simulink model "simulation"  (R2026b)
settings: Solver=ode23s  StopTime=T_sim  MaxStep=1e-3  MinStep=1e-7  RelTol=1e-5
InitFcn:
  | run param_file.m
values from neighbouring files (symbols this model uses):
  param = struct()    [param_file.m]    (also in param_file_2.m)
settings Model: Creator=user  LastModifiedBy=mahmu
settings SolverCC: ZeroCrossAlgorithm=Adaptive
settings DebuggingCC: IgnoredZcDiagnostic=none
settings SimscapeCC: SimscapeUseEnergyAccounting=off

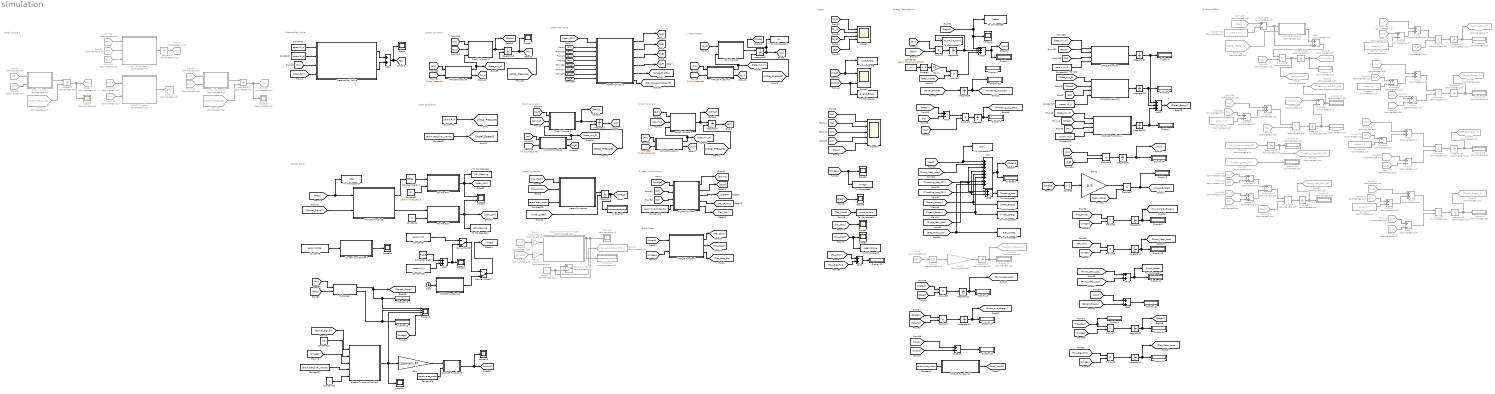
== system simulation ==
  note: Hydraulic Effort
  note: Small Volume A
  note: Control Policy
  note: BLDC Motor
  note: Energy Calculations
  note: Pressure Rail Valve
  note: Scope
  note: Initial Conditions
  note: Hydraulic Motor/Pump
  note: Inertia Dynamics
  note: Small Volume T
  note: Small Volume P
  note: Soft-Switch Valve
  note: Linear Actuator
  note: Small Voume A
  Add : Sum  Inputs=++++++++
  Add1 : Sum  Inputs=+-
  Add{10,12..13,15,17..18} (6 alike) : Sum  Commented=on
  Add11 : Sum  Commented=on  Inputs=+-
  Add14 : Sum  Commented=on  Inputs=+-
  Add16 : Sum  Commented=on  Inputs=+-
  Add2 : Sum  Inputs=+++
  Add{3..7,9} (6 alike) : Sum
  Add8 : Sum  Inputs=+++
  Clock : Clock
  Constant{,12,14..17} (6 alike) : Constant  Commented=on  Value=param.P_T
  Constant1 : Constant  Value=param.P_M
  Constant10 : Constant
  Constant11 : Constant  Value=15
  Constant13 : Constant  Value=param.P_M
  Constant18 : Constant  Value=param.VA_0
  Constant19 : Constant  Value=param.VP_0
  Constant2 : Constant  Value=param.P_H
  Constant20 : Constant  Value=param.VT_0
  Constant21 : Constant  Value=param.start_final_velocity
  Constant22 : Constant  Value=param.start_final_velocity
  Constant23 : Constant  Value=param.hyd_motor_fric
  Constant24 : Constant  Commented=on  Value=0
  Constant25 : Constant  Value=param.elec_motor
  Constant26 : Constant  Value=param.elec_motor
  Constant3 : Constant  Value=param.start_final_velocity
  Constant4 : Constant  Value=param.elec_motor
  Constant5 : Constant  Value=param.initial_stroke
  Constant6 : Constant  Value=0
  Constant7 : Constant  Value=param.P_M
  Constant8 : Constant  Value=param.stroke
  Constant9 : Constant  Value=param.P_H
  Display{,1..20,32,35..36} (24 alike) : Display
  Display{21..31,34} (12 alike) : Display  Commented=on
  Dynamics of Orifice 3 : Subsystem
  Electric Torque Controller1 : MATLAB Function  TreatAsAtomicUnit=on
  Experimental Friction Model : MATLAB Function  Commented=on  TreatAsAtomicUnit=on
  For the PRV : Subsystem
  For the SSV : Subsystem
  From : From  Commented=on  GotoTag=Initial_Pressure
  From100 : From  Commented=on  GotoTag=Q_A
  From{6,97,99,104} (4 alike) : From  Commented=on  GotoTag=Qh1
  From105 : From  Commented=on  GotoTag=Ph1
  From{98,106,113,133} (4 alike) : From  Commented=on  GotoTag=PA
  From112 : From  Commented=on  GotoTag=W_A
  From{21,114,134,168} (4 alike) : From  Commented=on  GotoTag=Q1
  From115 : From  Commented=on  GotoTag=Q_A
  From116 : From  Commented=on  GotoTag=Q_B
  From117 : From  Commented=on  GotoTag=PX
  From118 : From  Commented=on  GotoTag=W_X
  From119 : From  Commented=on  GotoTag=W_P
  From120 : From  Commented=on  GotoTag=PP
  From121 : From  Commented=on  GotoTag=Q_P
  From122 : From  Commented=on  GotoTag=Qpump
  From123 : From  Commented=on  GotoTag=PT
  From124 : From  Commented=on  GotoTag=W_T
  From125 : From  Commented=on  GotoTag=Pdes
  From126 : From  Commented=on  GotoTag=Qpump
  From127 : From  Commented=on  GotoTag=Q_T
  From128 : From  Commented=on  GotoTag=Input_HE
  From130 : From  Commented=on  GotoTag=W_A
  From131 : From  Commented=on  GotoTag=Initial_Pressure
  From135 : From  Commented=on  GotoTag=Throttling_Loss_SSV
  From140 : From  Commented=on  GotoTag=SSV_Power_throttle_HE
  From15 : From  Commented=on  GotoTag=PX
  From150 : From  Commented=on  GotoTag=Qleak
  From151 : From  Commented=on  GotoTag=PT
  From152 : From  Commented=on  GotoTag=PP
  From153 : From  Commented=on  GotoTag=W_P
  From154 : From  Commented=on  GotoTag=W_T
  From16 : From  Commented=on  GotoTag=omega
  From19 : From  Commented=on  GotoTag=Initial_Pressure
  From96 : From  Commented=on  GotoTag=Ph1
  Gain : Gain  Gain=1/param.Kt
  Gain1 : Gain  Gain=0.5
  Gain2 : Gain  Commented=on  Gain=0.000145038
  Gain3 : Gain  Commented=on  Gain=(60/(2*pi))
  Gain5 : Gain  Gain=0.5
  Gain6 : Gain  Commented=on  Gain=param.ResistHose
  Goto2 : Goto  Commented=on  GotoTag=Ph1
  Goto22 : Goto  Commented=on  GotoTag=experimental_friction
  Goto39 : Goto  Commented=on  GotoTag=PA
  Goto40 : Goto  Commented=on  GotoTag=Hose_Throttle_Loss
  Goto41 : Goto  Commented=on  GotoTag=Qh1
  Goto42 : Goto  Commented=on  GotoTag=Qh1
  Goto48 : Goto  Commented=on  GotoTag=Input_HE
  Goto49 : Goto  Commented=on  GotoTag=Stored_Energy_A
  Goto51 : Goto  Commented=on  GotoTag=Throttling_Loss_PRV_HE
  Goto52 : Goto  Commented=on  GotoTag=Throttling_Loss_SSV_HE
  Goto53 : Goto  Commented=on  GotoTag=Output_Energy
  Goto54 : Goto  Commented=on  GotoTag=Stored_Energy_P
  Goto55 : Goto  Commented=on  GotoTag=Stored_Energy_T
  Goto56 : Goto  Commented=on  GotoTag=Pump_Leak_Loss_HE
  Goto57 : Goto  Commented=on  GotoTag=Input_Power
  Hydraulic Motor : MATLAB Function  TreatAsAtomicUnit=on
  Inertia Dynamics : MATLAB Function  TreatAsAtomicUnit=on
  Integrator : Integrator  Commented=on  InitialConditionSource=external
  Integrator{1..4,18} (5 alike) : Integrator  InitialConditionSource=external
  Integrator{5,7..14,27..29,31} (13 alike) : Integrator
  Integrator{15,17,19..26} (10 alike) : Integrator  Commented=on
  Integrator16 : Integrator  Commented=on  InitialConditionSource=external
  MATLAB Function : MATLAB Function  TreatAsAtomicUnit=on
  MATLAB Function1 : MATLAB Function  TreatAsAtomicUnit=on
  MATLAB Function10 : MATLAB Function  TreatAsAtomicUnit=on
  MATLAB Function11 : MATLAB Function  TreatAsAtomicUnit=on
  MATLAB Function12 : MATLAB Function  TreatAsAtomicUnit=on
  MATLAB Function13 : MATLAB Function  TreatAsAtomicUnit=on
  MATLAB Function14 : MATLAB Function  TreatAsAtomicUnit=on
  MATLAB Function2 : MATLAB Function  Commented=on  TreatAsAtomicUnit=on
  MATLAB Function3 : MATLAB Function  TreatAsAtomicUnit=on
  MATLAB Function4 : MATLAB Function  Commented=on  TreatAsAtomicUnit=on
  MATLAB Function5 : MATLAB Function  TreatAsAtomicUnit=on
  MATLAB Function6 : MATLAB Function  TreatAsAtomicUnit=on
  MATLAB Function7 : MATLAB Function  TreatAsAtomicUnit=on
  MATLAB Function8 : MATLAB Function  TreatAsAtomicUnit=on
  MATLAB Function9 : MATLAB Function  Commented=on  TreatAsAtomicUnit=on
  Main Chamber : MATLAB Function  TreatAsAtomicUnit=on
  Manual Switch : ManualSwitch  CurrentSetting=0
  Manual Switch2 : ManualSwitch  CurrentSetting=0
  Manual Switch3 : ManualSwitch  Commented=on  CurrentSetting=0
  Pressure Rail Valve : MATLAB Function  TreatAsAtomicUnit=on
  Product{,1..8,16..17} (11 alike) : Product
  Product{9..15} (7 alike) : Product  Commented=on
  Pulse Generator : DiscretePulseGenerator  PulseType=Time based  Amplitude=param.P_H-param.P_M  Period=param.T_period  PulseWidth=50  PhaseDelay=param.delay
  Scope{,5..8,10..12,14..15,17} (11 alike) : Scope
      Scope settings: ActiveDisplayYMinimum=-7.8990948168927051E-6  ActiveDisplayYMaximum=6.46174239346027E-5  DataLoggingVariableName=ScopeData14
      Scope10 settings: ActiveDisplayYMinimum=-1  ActiveDisplayYMaximum=1  DataLoggingVariableName=ScopeData9
      Scope11 settings: ActiveDisplayYMinimum=-0.9375  ActiveDisplayYMaximum=0.9375  DataLoggingVariableName=ScopeData10
      Scope12 settings: ActiveDisplayYMinimum=-1  ActiveDisplayYMaximum=1  DataLoggingVariableName=ScopeData11
      Scope14 settings: ActiveDisplayYMinimum=-2.6515706692780068  ActiveDisplayYMaximum=0.29461896325311182  DataLoggingVariableName=ScopeData13
      Scope15 settings: ActiveDisplayYMinimum=-1  ActiveDisplayYMaximum=1  DataLoggingVariableName=ScopeData15
      Scope17 settings: ActiveDisplayYMinimum=2.5851457116932129E+6  ActiveDisplayYMaximum=1.1203688594761087E+7  DataLoggingVariableName=ScopeData17
      Scope5 settings: ActiveDisplayYMinimum=-714867.26768483547  ActiveDisplayYMaximum=268797.57913288096  DataLoggingVariableName=ScopeData3
      Scope6 settings: ActiveDisplayYMinimum=-2.1163885820684094E-7  ActiveDisplayYMaximum=1.4152197079471591E-6  DataLoggingVariableName=ScopeData5
      Scope7 settings: ActiveDisplayYMinimum=-1.2648949471331186  ActiveDisplayYMaximum=0.69609943857034651  DataLoggingVariableName=ScopeData6
      Scope8 settings: ActiveDisplayYMinimum=-1  ActiveDisplayYMaximum=1  DataLoggingVariableName=ScopeData7
  Scope1 : Scope  NumInputPorts=4
      settings: ActiveDisplayYMinimum=-0.00094060960760663083  ActiveDisplayYMaximum=0.00094060960760663083
  Scope13 : Scope  NumInputPorts=4
      settings: ActiveDisplayYMinimum=-0.12499999999999997  ActiveDisplayYMaximum=1.125  DataLoggingVariableName=ScopeData12
  Scope16 : Scope  Commented=on
      settings: ActiveDisplayYMinimum=2.3595705734494529E+6  ActiveDisplayYMaximum=1.140070781407249E+7  DataLoggingVariableName=ScopeData16
  Scope18 : Scope  Commented=on
      settings: ActiveDisplayYMinimum=2.6611575254358238E+8  ActiveDisplayYMaximum=4.6611575254358238E+8  DataLoggingVariableName=ScopeData18
  Scope2 : Scope  NumInputPorts=2
      settings: ActiveDisplayYMinimum=0.33341582524675561  ActiveDisplayYMaximum=8.9612181068995049
  Scope3 : Scope  NumInputPorts=5
      settings: ActiveDisplayYMinimum=1.6778033246308342E+6  ActiveDisplayYMaximum=1.9369768489858452E+7  DataLoggingVariableName=ScopeData2
  Scope4 : Scope  Commented=on
      settings: ActiveDisplayYMinimum=2.181490968537122E+6  ActiveDisplayYMaximum=1.1231186415855616E+7  DataLoggingVariableName=ScopeData4
  Scope9 : Scope  NumInputPorts=2
      settings: ActiveDisplayYMinimum=-2.9871968388761352  ActiveDisplayYMaximum=1.7269260169317651  DataLoggingVariableName=ScopeData8
  Small Volume A : MATLAB Function  Commented=on  TreatAsAtomicUnit=on
  Small Volume A1 : MATLAB Function  Commented=on  TreatAsAtomicUnit=on
  Small Volume A2 : MATLAB Function  TreatAsAtomicUnit=on
  Small Volume P : MATLAB Function  TreatAsAtomicUnit=on
  Small Volume T : MATLAB Function  TreatAsAtomicUnit=on
  Soft-switch Valve : MATLAB Function  TreatAsAtomicUnit=on
  Square : Math  Commented=on  Operator=square
  Square1 : Math  Operator=square
  Square5 : Math  Operator=square
  Subsystem : Subsystem
  Subtract : Sum  Inputs=+-
  Subtract{3,6..11,14} (8 alike) : Sum  Commented=on  Inputs=+-
  Subtract12 : Sum  Commented=on
  Subtract13 : Sum  Commented=on
  To Workspace : ToWorkspace  VariableName=Input_Energy  SaveFormat=Timeseries  SampleTime=-1
  To Workspace1 : ToWorkspace  VariableName=Output_Energy  SaveFormat=Timeseries  SampleTime=-1
  To Workspace10 : ToWorkspace  VariableName=PRV_Opening  SaveFormat=Timeseries  SampleTime=-1
  To Workspace11 : ToWorkspace  VariableName=SSV_Opening  SaveFormat=Timeseries  SampleTime=-1
  To Workspace12 : ToWorkspace  VariableName=Hydraulic_Input  SaveFormat=Timeseries  SampleTime=-1
  To Workspace13 : ToWorkspace  VariableName=Px  SaveFormat=Timeseries  SampleTime=-1
  To Workspace14 : ToWorkspace  VariableName=Pdes  SaveFormat=Timeseries  SampleTime=-1
  To Workspace15 : ToWorkspace  VariableName=regen_torque  SaveFormat=Timeseries  SampleTime=-1
  To Workspace16 : ToWorkspace  VariableName=pump_torque  SaveFormat=Timeseries  SampleTime=-1
  To Workspace2 : ToWorkspace  VariableName=Work  SaveFormat=Timeseries  SampleTime=-1
  To Workspace3 : ToWorkspace  VariableName=Throttling_Loss  SaveFormat=Timeseries  SampleTime=-1
  To Workspace4 : ToWorkspace  VariableName=Stored_Energy  SaveFormat=Timeseries  SampleTime=-1
  To Workspace5 : ToWorkspace  VariableName=Kinetic_Energy  SaveFormat=Timeseries  SampleTime=-1
  To Workspace6 : ToWorkspace  VariableName=omega  SaveFormat=Timeseries  SampleTime=-1
  To Workspace7 : ToWorkspace  VariableName=Pump_Losses  SaveFormat=Timeseries  SampleTime=-1
  To Workspace8 : ToWorkspace  VariableName=Elec_Losses  SaveFormat=Timeseries  SampleTime=-1
  To Workspace9 : ToWorkspace  VariableName=Regen  SaveFormat=Timeseries  SampleTime=-1
  Transport Delay2 : TransportDelay  DelayTime=param.delay_switch  InitialOutput=param.initial_stroke  BufferSize=1024*105
  wires:
  Constant2/1 -> Pressure Rail Valve/1(P)
  Small Volume A/1(Ph1dot) -> Integrator/1
  Constant1/1 -> [Initial_Pressure]
  From/1 -> Integrator/2
  Integrator/1 -> Goto2/1, Scope4/1  "PA"
  Small Volume P/1(PPdot) -> [PPdot], Integrator1/1
  [Initial_Pressure] -> Integrator1/2
  Small Volume T/1(PTdot) -> [PTdot], Integrator2/1
  [Initial_Pressure] -> Integrator2/2
  Main Chamber/1(PXdot) -> Integrator3/1
  [Initial_Pressure] -> Integrator3/2
  Integrator3/1 -> [PX], [PXdot], To Workspace13/1  "PX"
  [PA] -> Soft-switch Valve/3(PA)
  [omega] -> Hydraulic Motor/1(omega)
  Integrator1/1 -> [PP]  "PP"
  Integrator2/1 -> [PT]  "PT"
  [PP] -> Soft-switch Valve/2(PP)
  [PT] -> Soft-switch Valve/5(PT)
  [PX] -> Soft-switch Valve/4(PB)
  Soft-switch Valve/4(Q_T) -> [Q_T]  "Q_T"
  Soft-switch Valve/3(Q_B) -> [Q_B]  "Q_B"
  Soft-switch Valve/2(Q_A) -> [Q_A]  "Q_A"
  [Q_T] -> Small Volume T/1(QT)
  Hydraulic Motor/1(Qpump) -> [Qpump]
  [Qpump] -> Small Volume T/2(Qpump)
  [Qpump] -> Small Volume P/2(Qpump)
  [Q_P] -> Small Volume P/1(QP)
  [Q_B] -> Main Chamber/1(QB)
  From99/1 -> Small Volume A/2(Qh1)
  Constant22/1 -> [Initial_Speed]
  From21/1 -> Small Volume A/1(Q1)
  [Q_P] -> Scope1/1
  [Q_A] -> Scope1/2
  [Q_B] -> Scope1/3
  [Q_T] -> Scope1/4
  [Q1] -> Product/1
  [Pdes] -> Product/2
  Product/1 -> Integrator5/1
  [Work] -> To Workspace2/1, Add/1
  [Kinetic_Energy] -> To Workspace5/1, Add/6
  Add/1 -> Display3/1, [Output]
  [PA] -> Add1/2
  Add1/1 -> Product2/1
  [Q1] -> Product2/2
  Product2/1 -> Integrator7/1
  Integrator7/1 -> [Throttling_Loss_PRV], Display4/1
  [Throttling_Loss_PRV] -> Add3/1, Add/3
  Soft-switch Valve/1(Q_P) -> [Q_P]  "Q_P"
  Soft-switch Valve/5(Power_throttle) -> [Power_throttle]
  Integrator27/1 -> Display6/1, Add2/1
  Integrator28/1 -> Add2/2, Display2/1
  Square5/1 -> Gain5/1
  [omega] -> Square5/1
  [Stored_Energy] -> To Workspace4/1, Add/5
  Add2/1 -> [Stored_Energy]
  [Input] -> Scope2/1, To Workspace/1  "Input"
  [Output] -> To Workspace1/1, Scope2/2  "Output"
  Integrator8/1 -> Display35/1, [Throttling_Loss_SSV]
  [Throttling_Loss_SSV] -> Add3/2, Add/4
  Add3/1 -> To Workspace3/1
  [PX] -> Scope3/4
  [omega] -> Product3/2
  [Tau_Pump] -> Product3/1
  Integrator9/1 -> [Pump_Mech_Energy], Display9/1
  Product3/1 -> Integrator9/1
  Hydraulic Motor/3(DeltaP) -> [DeltaP]
  [DeltaP] -> Product4/1
  [Qpump] -> Product4/2
  Product4/1 -> Integrator10/1
  Integrator10/1 -> [Pump_Hyd_Energy], Display10/1
  [omega] -> To Workspace6/1, Scope5/1
  Hydraulic Motor/2(Qleak) -> [Qleak]
  [Qleak] -> Scope6/1
  [PT] -> Hydraulic Motor/2(PT)
  [PP] -> Hydraulic Motor/3(PP)
  [DeltaP] -> Product5/1
  [Qleak] -> Product5/2
  Product5/1 -> Integrator11/1
  Integrator11/1 -> [Pump_Leak_Loss], Display11/1
  [Pump_Mech_Loss] -> Add/2
  [Tau_fric] -> Product6/1
  [omega] -> Product6/2
  Product6/1 -> Integrator12/1
  Integrator12/1 -> [Pump_Mech_Loss], Display13/1
  [Pump_Leak_Loss] -> Add/7
  [Pump_Leak_Loss] -> Add5/1
  [Pump_Mech_Loss] -> Add5/2
  Add5/1 -> To Workspace7/1, Display14/1
  [Work] -> Add4/1
  [Stored_Energy] -> Add4/2
  Add4/1 -> Display12/1
  [Pdes] -> Scope3/5
  [PT] -> Scope3/3
  [PP] -> Scope3/2
  [omega] -> MATLAB Function1/2(omega)
  [current] -> MATLAB Function1/1(current)
  MATLAB Function1/1(Tau_Elec) -> [Tau_Elec]
  MATLAB Function1/2(Tau_Mech) -> [Tau_Mech]
  [Tau_Elec] -> Scope7/1
  [Tau_Mech] -> To Workspace15/1, Scope8/1
  For the PRV/1(Spool Opening) -> [open_PRV], To Workspace10/1, Scope9/1
  [Control_Signal] -> MATLAB Function3/2(Control_signal)
  Transport Delay2/1 -> For the PRV/1(Opening)
  MATLAB Function3/1(open_PRV) -> Transport Delay2/1
  MATLAB Function3/2(open_SSV) -> For the SSV/1(Opening)
  Pressure Rail Valve/1(Q_PA) -> Add6/1
  Pressure Rail Valve/2(Q_AT) -> Add6/2
  Add6/1 -> Scope/1, [Q1]
  [PA] -> Pressure Rail Valve/3(PA)
  Constant7/1 -> Pressure Rail Valve/2(T)
  [open_PRV] -> Pressure Rail Valve/4(spool_position)
  [open_SSV] -> Soft-switch Valve/1(spool_position)
  [Pdes] -> Subsystem/2(Pdes)
  [PX] -> Subsystem/1(PX)
  Subsystem/1(Control_Signal) -> [Control_Signal], Scope13/1, Display15/1  "Control Signal"
  Subsystem/2(delP) -> Scope13/2, Display16/1  "delP"
  Manual Switch2/1 -> [Pdes]  "Pdes"
  Constant10/1 -> Electric Torque Controller1/5(T_elec_max)
  Constant9/1 -> Manual Switch/1
  Constant13/1 -> Add7/2
  Pulse Generator/1 -> Add7/1
  Add7/1 -> Manual Switch/2, Scope12/1
  Dynamics of Orifice 3/1(Spool Opening) -> Scope10/1
  Constant8/1 -> Dynamics of Orifice 3/1(Stroke)
  [omega] -> Scope13/4
  [Control_Signal] -> Electric Torque Controller1/1(Control_Signal)
  Electric Torque Controller1/1(T_elec) -> Scope13/3, Gain/1, Scope11/1  "T_elec"
  [Pdes] -> To Workspace14/1, MATLAB Function3/1(Pdes)
  [Tau_Elec] -> Product7/1, Display5/1
  [omega] -> Product7/2
  Product7/1 -> Integrator13/1
  Integrator13/1 -> [Regen], Display17/1
  [Input] -> Subtract/1  "Input"
  [Output] -> Subtract/2  "Output"
  Subtract/1 -> Display18/1
  MATLAB Function1/3(Tau_Elec_Fric) -> [Tau_Elec_Fric]
  [Tau_Elec_Fric] -> Product8/1
  [omega] -> Product8/2
  Product8/1 -> Integrator14/1
  Integrator14/1 -> [Elec_Motor_Loss], Display19/1
  [Power_throttle] -> Integrator8/1
  [Pdes] -> Add1/1
  [Regen] -> To Workspace9/1, Add8/1, Scope14/1
  Integrator5/1 -> To Workspace12/1, Add8/2
  Add8/1 -> Display/1, [Input]
  [Elec_Motor_Loss] -> To Workspace8/1, Add/8
  [Initial_Speed] -> Integrator4/2
  Inertia Dynamics/1(omegadot) -> Integrator4/1
  Integrator4/1 -> Display32/1, [omega]  "omega"
  Gain/1 -> MATLAB Function13/1(current_in)
  MATLAB Function13/1(current) -> Scope15/1, [current]
  [Tau_Elec_Fric] -> Add9/2
  [Tau_fric] -> Add9/1
  Add9/1 -> Display20/1
  Constant5/1 -> For the PRV/2(Initial Stroke)
  Constant6/1 -> For the SSV/2(Initial Stroke)
  From6/1 -> Square/1
  Square/1 -> Gain6/1
  Gain6/1 -> Integrator15/1
  Integrator16/1 -> Scope16/1, Goto39/1  "PA"
  From19/1 -> Integrator16/2
  Small Volume A1/1(PAdot) -> Integrator16/1
  From97/1 -> Small Volume A1/1(Qh1)
  From100/1 -> Small Volume A1/2(QA)
  From96/1 -> MATLAB Function2/1(Ph1)
  From98/1 -> MATLAB Function2/2(PA)
  Integrator15/1 -> Goto40/1, Display22/1
  MATLAB Function2/1(Qh1dot) -> Integrator17/1
  Integrator17/1 -> Goto41/1
  From104/1 -> MATLAB Function2/3(Qh1)
  From105/1 -> MATLAB Function4/1(Ph1)
  From106/1 -> MATLAB Function4/2(PA)
  MATLAB Function4/1(Qh1) -> Goto42/1
  [Q_A] -> Small Volume A2/2(QA)
  Integrator18/1 -> [PA], Scope17/1  "PA"
  [Initial_Pressure] -> Integrator18/2
  Small Volume A2/1(PAdot) -> [PAdot], Integrator18/1
  MATLAB Function5/1(beta_mix_A) -> Small Volume A2/3(beta_mix), [beta_mix_A]
  [PA] -> MATLAB Function5/1(P)
  [PP] -> MATLAB Function6/1(P)
  MATLAB Function6/1(beta_mix) -> [beta_mix_P], Small Volume P/3(beta_mix)
  [PT] -> MATLAB Function7/1(P)
  MATLAB Function8/1(beta_mix) -> [beta_mix_X], Main Chamber/2(beta_mix)
  [PX] -> MATLAB Function8/1(P)
  MATLAB Function5/2(WA) -> [W_A]
  From113/1 -> Subtract3/1
  Constant/1 -> Subtract3/2
  Integrator19/1 -> Goto49/1, Display23/1
  From112/1 -> Add10/1
  Subtract3/1 -> Add10/2
  Add10/1 -> Product9/1
  Product9/1 -> Integrator19/1
  From115/1 -> Add11/2
  Add11/1 -> Product9/2
  MATLAB Function8/2(WX) -> [W_X]
  From117/1 -> Subtract6/1
  Constant12/1 -> Subtract6/2
  From118/1 -> Add12/1
  Subtract6/1 -> Add12/2
  Add12/1 -> Product10/1
  From116/1 -> Product10/2
  Product10/1 -> Integrator20/1
  Integrator20/1 -> Display24/1, Goto53/1
  MATLAB Function6/2(WP) -> [W_P]
  Constant14/1 -> Subtract8/2
  From120/1 -> Subtract8/1
  From119/1 -> Add13/1
  Subtract8/1 -> Add13/2
  From121/1 -> Add14/1
  From122/1 -> Add14/2
  Add13/1 -> Product11/1
  Add14/1 -> Product11/2
  Product11/1 -> Integrator21/1
  Integrator21/1 -> Goto54/1, Display25/1
  MATLAB Function7/2(WT) -> [W_T]
  Constant15/1 -> Subtract7/2
  From123/1 -> Subtract7/1
  Subtract7/1 -> Add15/2
  From124/1 -> Add15/1
  From126/1 -> Add16/1
  From127/1 -> Add16/2
  Add15/1 -> Product12/1
  Add16/1 -> Product12/2
  Product12/1 -> Integrator22/1
  Integrator22/1 -> Goto55/1, Display26/1
  From125/1 -> Subtract9/1
  Constant16/1 -> Subtract9/2
  MATLAB Function9/1(Win) -> Add17/1
  Subtract9/1 -> Add17/2, MATLAB Function9/1(P)
  Add17/1 -> Product13/1
  Product13/1 -> Goto57/1, Integrator23/1
  Integrator23/1 -> Goto48/1, Display28/1
  From131/1 -> MATLAB Function9/2(P_initial)
  [Initial_Pressure] -> MATLAB Function5/2(P_initial)
  Product14/1 -> Integrator24/1
  Add18/1 -> Product14/1
  Subtract10/1 -> Add18/2
  From130/1 -> Add18/1
  Integrator24/1 -> Subtract11/2, Display27/1
  Constant17/1 -> Subtract10/2
  From133/1 -> Subtract10/1
  From128/1 -> Subtract11/1
  Subtract11/1 -> Goto51/1, Display29/1
  [W_A] -> Soft-switch Valve/6(WA)
  [W_P] -> Soft-switch Valve/7(WP)
  [W_T] -> Soft-switch Valve/9(WT)
  [W_X] -> Soft-switch Valve/8(WB)
  Soft-switch Valve/6(SSV_Power_throttle_HE) -> [SSV_Power_throttle_HE]
  From140/1 -> Integrator25/1
  Integrator25/1 -> Goto52/1, Display30/1
  From135/1 -> Display31/1
  From150/1 -> Product15/2
  Product15/1 -> Integrator26/1
  From153/1 -> Subtract12/1
  From152/1 -> Subtract12/2
  From151/1 -> Subtract13/2
  From154/1 -> Subtract13/1
  Subtract12/1 -> Subtract14/1
  Subtract13/1 -> Subtract14/2
  Subtract14/1 -> Product15/1
  Integrator26/1 -> Goto56/1, Display34/1
  [Initial_Pressure] -> MATLAB Function8/2(P_initial)
  [Initial_Pressure] -> MATLAB Function6/2(P_initial)
  [Initial_Pressure] -> MATLAB Function7/2(P_initial)
  From168/1 -> Product13/2
  [Q1] -> Small Volume A2/1(Q1)
  From114/1 -> Add11/1
  From134/1 -> Product14/2
  [beta_mix_A] -> MATLAB Function/1(beta_mix)
  [PAdot] -> MATLAB Function/2(Pdot)
  [PA] -> MATLAB Function/3(P)
  Constant18/1 -> MATLAB Function/4(Volume)
  MATLAB Function/1(Stored_Power) -> Integrator27/1
  MATLAB Function10/1(Stored_Power) -> Integrator28/1
  [beta_mix_P] -> MATLAB Function10/1(beta_mix)
  [PPdot] -> MATLAB Function10/2(Pdot)
  [PP] -> MATLAB Function10/3(P)
  Constant19/1 -> MATLAB Function10/4(Volume)
  Integrator29/1 -> Add2/3, Display7/1
  MATLAB Function11/1(Stored_Power) -> Integrator29/1
  MATLAB Function7/1(beta_mix) -> [beta_mix_T], Small Volume T/3(beta_mix)
  [beta_mix_T] -> MATLAB Function11/1(beta_mix)
  [PTdot] -> MATLAB Function11/2(Pdot)
  [PT] -> MATLAB Function11/3(P)
  Constant20/1 -> MATLAB Function11/4(Volume)
  [Q_B] -> Product16/2
  [PX] -> Product16/1
  Product16/1 -> Integrator31/1
  Integrator31/1 -> Display36/1, [Work]
  [PA] -> Scope3/1
  [omega] -> Electric Torque Controller1/3(omega)
  Constant11/1 -> Electric Torque Controller1/2(Kp)
  Constant21/1 -> Electric Torque Controller1/4(start_final_velocity)
  Square1/1 -> Gain1/1
  Constant3/1 -> Square1/1
  Hydraulic Motor/4(Tau_Pump) -> [Tau_Pump]
  Hydraulic Motor/5(Tau_Fric) -> [Tau_fric]
  [Tau_Pump] -> Inertia Dynamics/2(Tau_Pump)
  Constant23/1 -> Hydraulic Motor/4(fric)
  Clock/1 -> MATLAB Function12/1(clock_time)
  MATLAB Function12/1(Pdes) -> Manual Switch2/2
  Manual Switch/1 -> Manual Switch2/1
  [Tau_Mech] -> Inertia Dynamics/1(Tau_Mech)
  From15/1 -> Gain2/1
  From16/1 -> Gain3/1
  Experimental Friction Model/1(friction) -> Display21/1, Manual Switch3/1, Scope18/1
  Gain2/1 -> Experimental Friction Model/1(pressure)
  Gain3/1 -> Experimental Friction Model/2(speed)
  Constant24/1 -> Goto22/1, Manual Switch3/2
  For the SSV/1(Spool Opening) -> [open_SSV], To Workspace11/1, Scope9/2
  Constant25/1 -> Inertia Dynamics/4(elec_motor)
  [Tau_Pump] -> To Workspace16/1
  Constant26/1 -> MATLAB Function13/2(elec_motor)
  Constant4/1 -> MATLAB Function14/1(elec_motor)
  MATLAB Function14/1(inertia) -> [total_inertia]
  Gain1/1 -> Product1/1
  [total_inertia] -> Product1/2
  Product1/1 -> Add8/3
  Gain5/1 -> Product17/1
  [total_inertia] -> Product17/2
  Product17/1 -> Display8/1, [Kinetic_Energy]

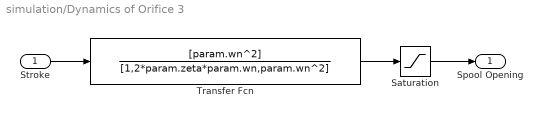
== system simulation/Dynamics of Orifice 3 ==
  Stroke : Inport
  Saturation : Saturate  UpperLimit=param.stroke  LowerLimit=0
  Transfer Fcn : TransferFcn  Numerator=[param.wn^2]  Denominator=[1,2*param.zeta*param.wn,param.wn^2]
  Spool Opening : Outport
  wires:
  Transfer Fcn/1 -> Saturation/1
  Saturation/1 -> Spool Opening/1
  Stroke/1 -> Transfer Fcn/1

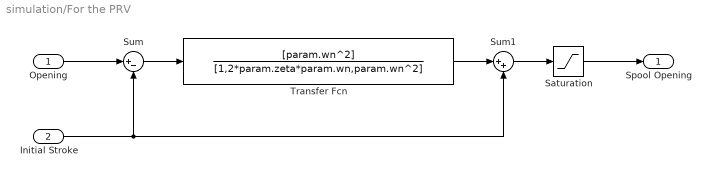
== system simulation/For the PRV ==
  Opening : Inport
  Initial Stroke : Inport  Port=2
  Saturation : Saturate  UpperLimit=1  LowerLimit=-1
  Sum : Sum  Inputs=|+-
  Sum1 : Sum  Inputs=|++
  Transfer Fcn : TransferFcn  Numerator=[param.wn^2]  Denominator=[1,2*param.zeta*param.wn,param.wn^2]
  Spool Opening : Outport
  wires:
  Saturation/1 -> Spool Opening/1
  Sum1/1 -> Saturation/1
  Transfer Fcn/1 -> Sum1/1
  Sum/1 -> Transfer Fcn/1
  Opening/1 -> Sum/1
  Initial Stroke/1 -> Sum1/2, Sum/2

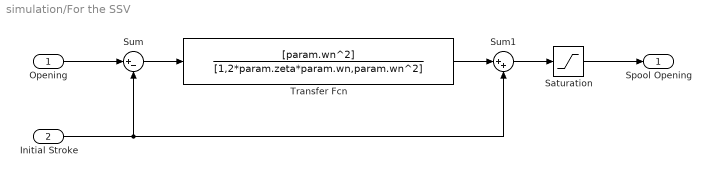
== system simulation/For the SSV ==
  Opening : Inport
  Initial Stroke : Inport  Port=2
  Saturation : Saturate  UpperLimit=1  LowerLimit=-1
  Sum : Sum  Inputs=|+-
  Sum1 : Sum  Inputs=|++
  Transfer Fcn : TransferFcn  Numerator=[param.wn^2]  Denominator=[1,2*param.zeta*param.wn,param.wn^2]
  Spool Opening : Outport
  wires:
  Saturation/1 -> Spool Opening/1
  Sum1/1 -> Saturation/1
  Transfer Fcn/1 -> Sum1/1
  Sum/1 -> Transfer Fcn/1
  Opening/1 -> Sum/1
  Initial Stroke/1 -> Sum1/2, Sum/2

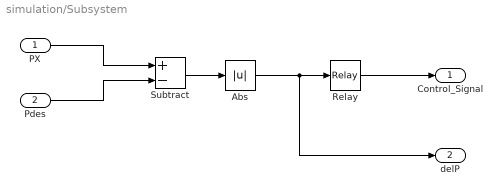
== system simulation/Subsystem ==
  PX : Inport
  Pdes : Inport  Port=2
  Abs : Abs  SaturateOnIntegerOverflow=off
  Relay : Relay  OnSwitchValue=15e5  OffSwitchValue=1e4  OnOutputValue=0  OffOutputValue=1
  Subtract : Sum  Inputs=+-
  Control_Signal : Outport
  delP : Outport  Port=2
  wires:
  PX/1 -> Subtract/1
  Pdes/1 -> Subtract/2
  Subtract/1 -> Abs/1
  Abs/1 -> delP/1, Relay/1
  Relay/1 -> Control_Signal/1

== matlab function simulation/Inertia Dynamics ==
  data: Tau_Mech input; Tau_Pump input; omegadot output; param parameter; experimental_friction input; elec_motor input
function omegadot  = Inertia_Dyn(Tau_Mech, Tau_Pump, param, experimental_friction, elec_motor)

if elec_motor == 1
    omegadot = (Tau_Pump + Tau_Mech - experimental_friction) / (param.J_hyd + param.J_elec);
elseif elec_motor == 0
    omegadot = (Tau_Pump + Tau_Mech - experimental_friction) / (param.J_hyd);
else
    omegadot = 0;
end

== matlab function simulation/MATLAB Function3 ==
  data: Pdes input; open_PRV output; open_SSV output; param parameter; Control_signal input
function [open_PRV, open_SSV] = fcn(Pdes, param, Control_signal)

if Pdes == param.P_H && Control_signal == 0
    open_PRV = 1;
    open_SSV = 1;

elseif Pdes == param.P_M && Control_signal == 0
    open_PRV = -1;
    open_SSV = -1;

elseif Pdes == param.P_H && Control_signal > 0
    open_PRV = 1;
    open_SSV = 0;

elseif Pdes == param.P_M && Control_signal > 0
    open_PRV = -1;
    open_SSV = 0;
    
else
    open_PRV = 0;
    open_SSV = 0;
end

== matlab function simulation/MATLAB Function9 ==
  data: P input; P_initial input; Win output; param parameter
function Win = oil_comp(P,P_initial,param)

Pg = P-param.P_T;   % Gauge pressure
r = P/param.P_T;    % Pressure ratio
e = exp(Pg/param.beta); 
rv = (1./e+param.air*r.^(-1/param.gamma))/(1+param.air);      %Volume ratio

El = param.beta*(e - (1 + Pg/param.beta)) + param.P_T*(e - 1);              % Energy in liquid
Eg = P/(param.gamma - 1) .* (1 - r.^(1/param.gamma - 1));           % Energy in gas
E  = (El./e + param.air*Eg.*r.^(-1/param.gamma)) ./ ...
     (1./e + param.air*r.^(-1/param.gamma));                       % Energy in mixture
Win  = E - (1./rv - 1)*P_initial;                                 % Compressibility energy density

== matlab function simulation/MATLAB Function1 ==
  data: current input; omega input; Tau_Elec output; param parameter; Tau_Mech output; Tau_Elec_Fric output
function [Tau_Elec, Tau_Mech, Tau_Elec_Fric] = BLDC(current, omega, param)

% Limit current to stall current
I_stall = 69;
current = min(max(current, -I_stall), I_stall);

% Electromagnetic torque
Tau_Elec = param.Kt * current;

% Friction torque (viscous model)
Tau_Elec_Fric = param.B * omega;

% Mechanical torque available at shaft
Tau_Mech = Tau_Elec - Tau_Elec_Fric;

end

== matlab function simulation/MATLAB Function2 ==
  data: Ph1 input; PA input; Qh1 input; Qh1dot output; param parameter
function Qh1dot = Small_Vol_A_Hose_Dynamics(Ph1, PA, Qh1, param)

Qh1dot = ((Ph1 - PA) - param.ResistHose*Qh1)/param.InertHose;

== matlab function simulation/Electric Torque Controller1 ==
  data: Control_Signal input; Kp input; omega input; T_elec output; start_final_velocity input; T_elec_max input; param parameter
% function T_elec  = fcn(Control_Signal, Kp, omega, start_final_velocity, T_elec_max, param)
% 
% if Control_Signal == 1 
% 
%     if omega < start_final_velocity
%         omega_error = omega -start_final_velocity;
%         T_elec = - (Kp*omega_error);
%     else
%         T_elec = -T_elec_max;
%     end
% 
% else
%     if omega >= param.max_speed-0.01
%         omega_error = omega - param.max_speed;
%         T_elec = -(Kp*omega_error);
%     else
%         T_elec = T_elec_max;
%     end
% 
% end

function T_elec = fcn(Control_Signal, Kp, omega, ...
    start_final_velocity, T_elec_max, param)

if Control_Signal == 1
    target_speed = start_final_velocity;
else
    target_speed = param.max_speed;
end

omega_error = omega - target_speed;

T_elec = -Kp * omega_error;

% Saturate torque
T_elec = min(max(T_elec, -T_elec_max), T_elec_max);

end

== matlab function simulation/Small Volume A1 ==
  data: Qh1 input; QA input; PAdot output; param parameter
function PAdot = Small_Vol_A(Qh1,QA, param)

PAdot = (param.beta/param.VA_0)*(Qh1-QA);

== matlab function simulation/MATLAB Function4 ==
  data: Ph1 input; PA input; Qh1 output; param parameter
function Qh1 = Small_Vol_A_Hose_Dynamics(Ph1, PA, param)

Qh1 = (Ph1 - PA)/param.ResistHose;

== matlab function simulation/Small Volume A2 ==
  data: Q1 input; PAdot output; QA input; beta_mix input; param parameter
function PAdot = Small_Vol_A(Q1,QA, beta_mix, param)

PAdot = (beta_mix/param.VA_0)*(Q1-QA);

== matlab function simulation/MATLAB Function5 ==
  data: P input; P_initial input; beta_mix_A output; param parameter; WA output
function [beta_mix_A, WA] = oil_comp(P,P_initial,param)

Pg = P-param.P_T;   % Gauge pressure
r = P/param.P_T;    % Pressure ratio
e = exp(Pg/param.beta); 
rv = (1./e+param.air*r.^(-1/param.gamma))/(1+param.air);      %Volume ratio

beta_mix_A = rv*(1+param.air)/(1/(e*param.beta)+...
           param.air/(param.gamma*param.P_T*r^(1/param.gamma+1)));

El = param.beta*(e - (1 + Pg/param.beta)) + param.P_T*(e - 1);              % Energy in liquid
Eg = P/(param.gamma - 1) .* (1 - r.^(1/param.gamma - 1));           % Energy in gas
E  = (El./e + param.air*Eg.*r.^(-1/param.gamma)) ./ ...
     (1./e + param.air*r.^(-1/param.gamma));                       % Energy in mixture
WA  = E - (1./rv - 1)*P_initial;                                 % Compressibility energy density

== matlab function simulation/MATLAB Function6 ==
  data: P input; P_initial input; beta_mix output; param parameter; WP output
function [beta_mix, WP] = oil_comp(P,P_initial,param)

%Ph=7e6, P0=1e5
Pg = P-param.P_T;   % Gauge pressure
r = P/param.P_T;    % Pressure ratio
e = exp(Pg/param.beta); 
rv = (1./e+param.air*r.^(-1/param.gamma))/(1+param.air);      %Volume ratio

beta_mix = rv*(1+param.air)/(1/(e*param.beta)+...
           param.air/(param.gamma*param.P_T*r^(1/param.gamma+1)));

El = param.beta*(e - (1 + Pg/param.beta)) + param.P_T*(e - 1);              % Energy in liquid
Eg = P/(param.gamma - 1) .* (1 - r.^(1/param.gamma - 1));           % Energy in gas
E  = (El./e + param.air*Eg.*r.^(-1/param.gamma)) ./ ...
     (1./e + param.air*r.^(-1/param.gamma));                       % Energy in mixture
WP  = E - (1./rv - 1)*P_initial;                                 % Compressibility energy density

== matlab function simulation/MATLAB Function7 ==
  data: P input; P_initial input; beta_mix output; param parameter; WT output
function [beta_mix, WT] = oil_comp(P,P_initial,param)

%Ph=7e6, P0=1e5
Pg = P-param.P_T;   % Gauge pressure
r = P/param.P_T;    % Pressure ratio
e = exp(Pg/param.beta); 
rv = (1./e+param.air*r.^(-1/param.gamma))/(1+param.air);      %Volume ratio

beta_mix = rv*(1+param.air)/(1/(e*param.beta)+...
           param.air/(param.gamma*param.P_T*r^(1/param.gamma+1)));


El = param.beta*(e - (1 + Pg/param.beta)) + param.P_T*(e - 1);              % Energy in liquid
Eg = P/(param.gamma - 1) .* (1 - r.^(1/param.gamma - 1));           % Energy in gas
E  = (El./e + param.air*Eg.*r.^(-1/param.gamma)) ./ ...
     (1./e + param.air*r.^(-1/param.gamma));                       % Energy in mixture
WT  = E - (1./rv - 1)*P_initial;                                 % Compressibility energy density

== matlab function simulation/Small Volume A ==
  data: Q1 input; Ph1dot output; Qh1 input; param parameter
function Ph1dot = Small_Vol_A(Q1,Qh1, param)

Ph1dot = (param.beta/param.VA_0)*(Q1-Qh1);

== matlab function simulation/MATLAB Function8 ==
  data: P input; P_initial input; beta_mix output; param parameter; WX output
function [beta_mix, WX] = oil_comp(P,P_initial,param)

%Ph=7e6, P0=1e5
Pg = P-param.P_T;   % Gauge pressure
r = P/param.P_T;    % Pressure ratio
e = exp(Pg/param.beta); 
rv = (1./e+param.air*r.^(-1/param.gamma))/(1+param.air);      %Volume ratio

beta_mix = rv*(1+param.air)/(1/(e*param.beta)+...
           param.air/(param.gamma*param.P_T*r^(1/param.gamma+1)));

El = param.beta*(e - (1 + Pg/param.beta)) + param.P_T*(e - 1);              % Energy in liquid
Eg = P/(param.gamma - 1) .* (1 - r.^(1/param.gamma - 1));           % Energy in gas
E  = (El./e + param.air*Eg.*r.^(-1/param.gamma)) ./ ...
     (1./e + param.air*r.^(-1/param.gamma));                       % Energy in mixture
WX  = E - (1./rv - 1)*P_initial;                                 % Compressibility energy density

== matlab function simulation/MATLAB Function ==
  data: beta_mix input; Stored_Power output; Pdot input; P input; Volume input
function Stored_Power = fcn(beta_mix, Pdot, P, Volume)

Stored_Power = P*(Volume/beta_mix)*Pdot;

== matlab function simulation/MATLAB Function10 ==
  data: beta_mix input; Stored_Power output; Pdot input; P input; Volume input
function Stored_Power = fcn(beta_mix, Pdot, P, Volume)

Stored_Power = P*(Volume/beta_mix)*Pdot;

== matlab function simulation/MATLAB Function11 ==
  data: beta_mix input; Stored_Power output; Pdot input; P input; Volume input
function Stored_Power = fcn(beta_mix, Pdot, P, Volume)

Stored_Power = P*(Volume/beta_mix)*Pdot;

== matlab function simulation/MATLAB Function12 ==
  data: clock_time input; Pdes output; param parameter
function Pdes = fcn(clock_time, param)

if clock_time > 0.2 && clock_time < 0.75
    Pdes = param.P_H;
else
    Pdes = param.P_M;
end

== matlab function simulation/Experimental Friction Model ==
  data: pressure input; friction output; speed input
function friction  = friction_model(pressure, speed)

C = [-2.7371712380878151e-20 -1.012140531055926e-17 1.362680380791501e-14 2.5017160289203132e-12;
    7.8175012770957013e-17 6.5819426994446848e-14 -5.7218700361030071e-11 -2.6554187394929447e-08;
    -3.0602563559828119e-14 -2.3014653747973892e-10 2.0537443634696756e-07 0.00011211247665566631;
    8.9217552784699898e-12 5.982060290372595e-08 7.3192331395694632e-05 0.083988065486528374];

p = [pressure^3; pressure^2; pressure; 1];
w = [speed^3; speed^2; speed; 1];

friction = sum((C * p) .* w);
end

== matlab function simulation/MATLAB Function13 ==
  data: current_in input; current output; elec_motor input
function current = fcn(current_in, elec_motor)

if elec_motor == 1
    current = current_in;
elseif elec_motor == 0
    current = 0;
else
    current = 0;
end

== matlab function simulation/MATLAB Function14 ==
  data: inertia output; elec_motor input; param parameter
function inertia = fcn(elec_motor, param)

if elec_motor == 1
    inertia = (param.J_hyd+param.J_elec);
elseif elec_motor == 0
    inertia = param.J_hyd;
else
    inertia = 0;
end

== matlab function simulation/Pressure Rail Valve ==
  data: P input; T input; Q_PA output; Q_AT output; PA input; spool_position input; param parameter
function [Q_PA, Q_AT] = RailValve(P, T, PA, spool_position, param)

db = param.valve_buffer;

spool_position = max(-1, min(1, spool_position));

if abs(spool_position) <= db
    f = 0;
else
    f = (abs(spool_position) - db) / (1 - db);
    f = max(0, min(1, f));
end

A_PA = 0;
A_AT = 0;

if spool_position > db
    A_PA = param.max_Avt * f;
elseif spool_position < -db
    A_AT = param.max_Avt * f;
end

Q_PA = param.Cd * A_PA * sqrt(2/param.rho) * sqrt(abs(P-PA)) * sign(P-PA);
Q_AT = param.Cd * A_AT * sqrt(2/param.rho) * sqrt(abs(PA-T)) * sign(T-PA);

end

== matlab function simulation/Soft-switch Valve ==
  data: spool_position input; Q_P output; PP input; PA input; PB input; PT input; Q_A output; Q_B output; Q_T output; param parameter; Power_throttle output; WA input; WP input; WB input; WT input; SSV_Power_throttle_HE output
function [Q_P, Q_A, Q_B, Q_T, Power_throttle, SSV_Power_throttle_HE] = SSV(spool_position, PP, PA, PB, PT, param, WA, WP, WB, WT)

db = 0.02; % spool deadband around zero (fraction of full stroke)

spool_position = max(-1, min(1, spool_position));

if abs(spool_position) <= db
    f = 0;
else
    f = (abs(spool_position) - db) / (1 - db);
    f = max(0, min(1, f));
end

A_PA = 0; A_PB = 0; A_AT = 0; A_BT = 0; A_PT = 0; A_AB = 0;

if abs(spool_position) <= db
    A_PT = param.max_Avt;
    A_AB = param.max_Avt;
elseif spool_position > 0
    A_PA = param.max_Avt * f;
    A_BT = param.max_Avt * f;
elseif spool_position < 0
    A_PB = param.max_Avt * f;
    A_AT = param.max_Avt * f;
end

Q_PA = param.Cd*A_PA*sign(PP-PA)*sqrt((2/param.rho)*abs(PP-PA));
Q_PB = param.Cd*A_PB*sign(PP-PB)*sqrt((2/param.rho)*abs(PP-PB));
Q_AT = param.Cd*A_AT*sign(PA-PT)*sqrt((2/param.rho)*abs(PA-PT));
Q_BT = param.Cd*A_BT*sign(PB-PT)*sqrt((2/param.rho)*abs(PB-PT));
Q_PT = param.Cd*A_PT*sign(PP-PT)*sqrt((2/param.rho)*abs(PP-PT));
Q_AB = param.Cd*A_AB*sign(PA-PB)*sqrt((2/param.rho)*abs(PA-PB));

Q_P = -(Q_PA + Q_PB + Q_PT);
Q_A =  Q_AT + Q_AB - Q_PA;
Q_B =  Q_BT - Q_AB - Q_PB;
Q_T =  -Q_PT - Q_AT - Q_BT;

Q_B = -Q_B;

PPg = PP - param.P_T;
PAg = PA - param.P_T;
PBg = PB - param.P_T;
PTg = PT - param.P_T;

SSV_Power_throttle_HE = ...
    abs(Q_PA)*abs((WP+PPg)-(WA+PAg)) + ...
    abs(Q_PB)*abs((WP+PPg)-(WB+PBg)) + ...
    abs(Q_AT)*abs((WA+PAg)-(WT+PTg)) + ...
    abs(Q_BT)*abs((WB+PBg)-(WT+PTg)) + ...
    abs(Q_PT)*abs((WP+PPg)-(WT+PTg)) + ...
    abs(Q_AB)*abs((WA+PAg)-(WB+PBg));

Power_throttle = ...
    abs(Q_PA)*abs(PP-PA) + ...
    abs(Q_PB)*abs(PP-PB) + ...
    abs(Q_AT)*abs(PA-PT) + ...
    abs(Q_BT)*abs(PB-PT) + ...
    abs(Q_PT)*abs(PP-PT) + ...
    abs(Q_AB)*abs(PA-PB);

end

== matlab function simulation/Small Volume P ==
  data: QP input; PPdot output; Qpump input; param parameter; beta_mix input
function PPdot = Small_Vol_P(QP,Qpump, param, beta_mix)

PPdot = (beta_mix/param.VP_0)*(QP-Qpump);

== matlab function simulation/Hydraulic Motor ==
  data: Qpump output; Qleak output; omega input; PT input; PP input; fric input; param parameter; DeltaP output; Tau_Pump output; Tau_Fric output
function [Qpump, Qleak, DeltaP, Tau_Pump, Tau_Fric] = Hyd_Motor(omega, PT, PP, fric, param)

    DeltaP = PP - PT;

    Tau_Ideal = (param.D/(2*pi)) * DeltaP;
    
    % Pump friction model
    if fric == 1
        Tau_fr_nom = ((1 - param.eta_m_nom)/param.eta_m_nom) ...
                      * (param.D/(2*pi)) * param.dp_nom;
        
        k = (Tau_fr_nom - param.tau0) / param.dp_nom;
        
        omega_nom_rad = 2*pi*param.omega_nom/60;
        
        s = tanh(4*omega/(5e-5*omega_nom_rad));
        
        Tau_Fric = (param.tau0 + k*abs(DeltaP)) * s;
    else
        Tau_Fric = 0;
    end

    Tau_Pump = Tau_Ideal - Tau_Fric;

    % Analytical leakage model (Simscape-equivalent)
    
    % Parameters
    D     = param.D;          
    eta_v = param.eta_v_nom;  % nominal volumetric efficiency
    omega_nom = param.omega_nom;      % [rad/s]
    DeltaP_nom = param.dp_nom;    % [Pa]
    rho   = param.rho;        % [kg/m^3]
    
    % Hagen–Poiseuille coefficient
    K = (D/(2*pi))*omega_nom*(1 - eta_v)/DeltaP_nom;
    
    % Mass leakage flow
    m_dot_leak = K * rho * DeltaP;
    
    % Convert to volumetric leakage
    Qleak = m_dot_leak / rho;
    
    % Ideal displacement flow
    Qideal = (D/(2*pi)) * omega;
    
    % Net flow (same convention as Simscape)
    Qpump = Qideal + Qleak;
end

== matlab function simulation/Small Volume T ==
  data: QT input; PTdot output; Qpump input; param parameter; beta_mix input
function PTdot = Small_Vol_T(QT,Qpump,param, beta_mix)

PTdot = (beta_mix/param.VT_0)*(Qpump-QT);

== matlab function simulation/Main Chamber ==
  data: QB input; PXdot output; param parameter; beta_mix input
function PXdot = Main_Chamber(QB, param, beta_mix)

PXdot = (beta_mix/param.V1_0)*(QB);
